simulink model "NIELITCombined_fixed"  (R2025a)
settings: Solver=ode45  StartTime=0.0  StopTime=100  MaxStep=2e-5  RelTol=1e-3
libraries: simulink x1
settings Model: Creator=naray  LastModifiedBy=naray

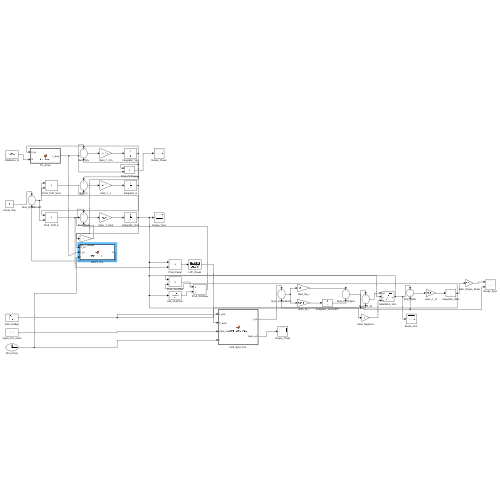
[thumbnail: Simulink's stored preview of the top-level diagram]
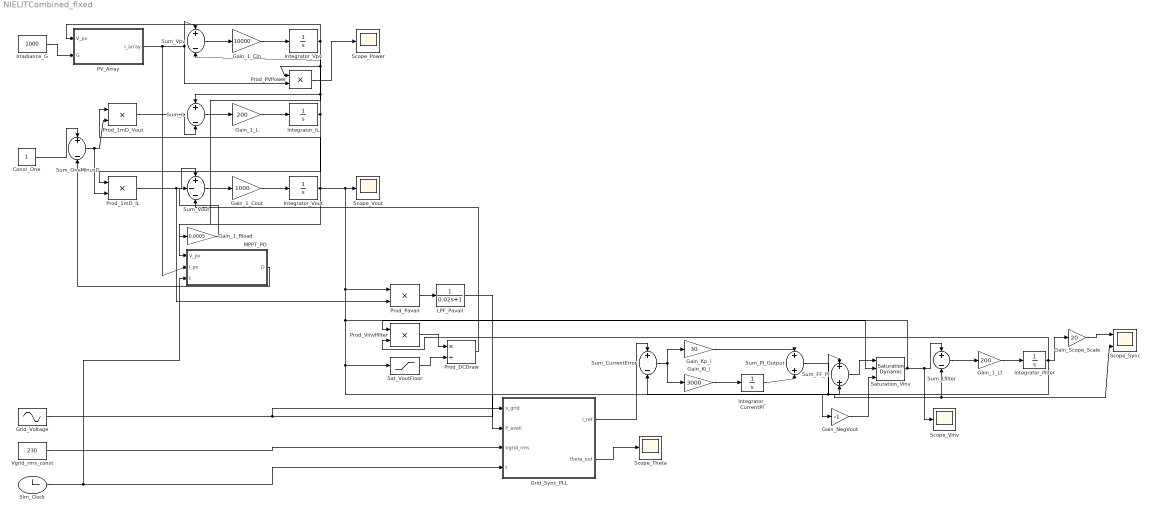
== system NIELITCombined_fixed ==
  Const_One : Constant
  Gain_1_Cin : Gain  Gain=10000
  Gain_1_Cout : Gain  Gain=1000
  Gain_1_L : Gain  Gain=200
  Gain_1_Lf : Gain  Gain=200
  Gain_1_Rload : Gain  Gain=0.0005
  Gain_Ki_i : Gain  Gain=3000
  Gain_Kp_i : Gain  Gain=30
  Gain_NegVout : Gain  Gain=-1
  Gain_Scope_Scale : Gain  Gain=20
  Grid_Sync_PLL : MATLAB Function  TreatAsAtomicUnit=on
  Grid_Voltage : Sin  Amplitude=325.2691  Frequency=314.1593  SampleTime=0
  Integrator_CurrentPI : Integrator
  Integrator_Vout : Integrator  InitialCondition=350
  Integrator_Vpv : Integrator  InitialCondition=300
  Integrator_iL : Integrator
  Integrator_ifilter : Integrator
  Irradiance_G : Constant  Value=1000
  LPF_Pavail : TransferFcn  Denominator=[0.02 1]
  MPPT_PO : MATLAB Function  TreatAsAtomicUnit=on
  PV_Array : MATLAB Function  TreatAsAtomicUnit=on
  Prod_1mD_Vout : Product
  Prod_1mD_iL : Product
  Prod_DCDraw : Product  Inputs=*/
  Prod_PVPower : Product
  Prod_Pavail : Product
  Prod_VinvIfilter : Product
  Sat_VoutFloor : Saturate  UpperLimit=1000  LowerLimit=50
  Saturation_Vinv : simulink/Discontinuities/Saturation Dynamic  OutMin=[]  OutMax=[]  OutDataTypeStr=Inherit: Same as second input  OutDataType=fixdt(1, 16)  OutScaling=2^-10  DoSatur=off
  Scope_Power : Scope
      settings: ActiveDisplayYMinimum=83.879513740278981  ActiveDisplayYMaximum=3287.1437398474195
  Scope_Sync : Scope  NumInputPorts=2
      settings: ActiveDisplayYMinimum=-448.184779047426  ActiveDisplayYMaximum=337.89270833968885
  Scope_Theta : Scope
      settings: ActiveDisplayYMinimum=-0.7853974821483809  ActiveDisplayYMaximum=7.0685802525916088
  Scope_Vinv : Scope
      settings: ActiveDisplayYMinimum=-415.88461066533625  ActiveDisplayYMaximum=415.4691551949615
  Scope_Vout : Scope
      settings: ActiveDisplayYMinimum=-1  ActiveDisplayYMaximum=1
  Sim_Clock : Clock
  Sum_CurrentError : Sum  Inputs=+-
  Sum_FF_PI : Sum
  Sum_Lfilter : Sum  Inputs=+-
  Sum_OneMinusD : Sum  Inputs=+-
  Sum_PI_Output : Sum
  Sum_Vout : Sum  Inputs=+--
  Sum_Vpv : Sum  Inputs=+-
  Sum_iL : Sum  Inputs=+-
  Vgrid_rms_const : Constant  Value=230
  wires:
  Irradiance_G/1 -> PV_Array/2(G)
  Integrator_Vpv/1 -> Sum_iL/1, MPPT_PO/1(V_pv), Prod_PVPower/1, PV_Array/1(V_pv)
  PV_Array/1(I_array) -> Sum_Vpv/1, Prod_PVPower/2, MPPT_PO/2(I_pv)
  Prod_PVPower/1 -> Scope_Power/1
  Integrator_iL/1 -> Sum_Vpv/2, Prod_1mD_iL/1
  Sum_Vpv/1 -> Gain_1_Cin/1
  Gain_1_Cin/1 -> Integrator_Vpv/1
  Prod_1mD_Vout/1 -> Sum_iL/2
  Sum_iL/1 -> Gain_1_L/1
  Gain_1_L/1 -> Integrator_iL/1
  Integrator_Vout/1 -> Gain_NegVout/1, Sat_VoutFloor/1, Saturation_Vinv/2, Prod_Pavail/1, Scope_Vout/1, Prod_1mD_Vout/1, Gain_1_Rload/1
  Sum_OneMinusD/1 -> Prod_1mD_Vout/2, Prod_1mD_iL/2
  Const_One/1 -> Sum_OneMinusD/1
  MPPT_PO/1(D) -> Sum_OneMinusD/2
  Prod_1mD_iL/1 -> Sum_Vout/1, Prod_Pavail/2
  Gain_1_Rload/1 -> Sum_Vout/2
  Prod_DCDraw/1 -> Sum_Vout/3
  Sum_Vout/1 -> Gain_1_Cout/1
  Gain_1_Cout/1 -> Integrator_Vout/1
  Grid_Voltage/1 -> Sum_Lfilter/2, Scope_Sync/2, Sum_FF_PI/1, Grid_Sync_PLL/1(v_grid)
  Prod_Pavail/1 -> LPF_Pavail/1
  LPF_Pavail/1 -> Grid_Sync_PLL/2(P_avail)
  Vgrid_rms_const/1 -> Grid_Sync_PLL/3(Vgrid_rms)
  Sim_Clock/1 -> Grid_Sync_PLL/4(t), MPPT_PO/3(t)
  Grid_Sync_PLL/1(i_ref) -> Sum_CurrentError/1
  Grid_Sync_PLL/2(theta_out) -> Scope_Theta/1
  Integrator_ifilter/1 -> Sum_CurrentError/2, Gain_Scope_Scale/1, Prod_VinvIfilter/2
  Sum_CurrentError/1 -> Gain_Kp_i/1, Gain_Ki_i/1
  Gain_Ki_i/1 -> Integrator_CurrentPI/1
  Gain_Kp_i/1 -> Sum_PI_Output/1
  Integrator_CurrentPI/1 -> Sum_PI_Output/2
  Sum_PI_Output/1 -> Sum_FF_PI/2
  Sum_FF_PI/1 -> Saturation_Vinv/1
  Gain_NegVout/1 -> Saturation_Vinv/3
  Saturation_Vinv/1 -> Scope_Vinv/1, Sum_Lfilter/1, Prod_VinvIfilter/1
  Sum_Lfilter/1 -> Gain_1_Lf/1
  Gain_1_Lf/1 -> Integrator_ifilter/1
  Gain_Scope_Scale/1 -> Scope_Sync/1
  Prod_VinvIfilter/1 -> Prod_DCDraw/1
  Sat_VoutFloor/1 -> Prod_DCDraw/2

== matlab function NIELITCombined_fixed/MPPT_PO ==
  settings: updateMethod=DISCRETE
  data: V_pv input; D output; I_pv input; t input
function D = MPPT_PO(V_pv, I_pv, t)
    persistent D_prev direction P_prev t_last
    if isempty(D_prev)
        D_prev = 0.5;      % your existing initial duty cycle
        direction = 1;
        P_prev = 0;
        t_last = -Inf;
    end

    Ts_mppt = 0.02;        % sample interval: ~4x the 20ms LPF time constant
    Dstep   = 0.005;       % consider halving your current step size too

    if (t - t_last) >= Ts_mppt
        P = V_pv * I_pv;
        if P < P_prev
            direction = -direction;
        end
        D_prev = D_prev + direction * Dstep;
        D_prev = min(max(D_prev, 0.05), 0.95);  % keep your existing D_min/D_max
        P_prev = P;
        t_last = t;
    end

    D = D_prev;   % hold last decision between updates
end

== matlab function NIELITCombined_fixed/PV_Array ==
  data: V_pv input; I_array output; G input
function I_array = PV_Array(V_pv, G)
% Simplified single-diode PV model for a 12-panel series STRING
Isc = 8.8; Voc = 444; n = 1.3; Ns = 720; Vt = 0.02585;
Iph = Isc * (G/1000);
Io  = Isc / (exp(Voc/(n*Vt*Ns)) - 1);
I_array = Iph - Io*(exp(V_pv/(n*Vt*Ns)) - 1);
I_array = max(I_array, 0);
end

== matlab function NIELITCombined_fixed/Grid_Sync_PLL ==
  settings: updateMethod=DISCRETE
  data: v_grid input; i_ref output; P_avail input; Vgrid_rms input; t input; theta_out output
function [i_ref, theta_out] = Grid_Sync_PLL(v_grid, P_avail, Vgrid_rms, t)
% SOGI-PLL (clock-based adaptive timing, vd-driven PI)
persistent x1 x2 theta integral_term t_prev
if isempty(x1)
    x1 = 0; x2 = 0; theta = 0; integral_term = 0; t_prev = 0;
end
dt = t - t_prev;
t_prev = t;
if dt <= 0
    dt = 1e-6;
end
k = 1.4142;
omega0 = 2*pi*50;
Kp_pll = 180;
Ki_pll = 3200;

x1_new = x1 + dt*omega0*(k*(v_grid - x1) - x2);
x2_new = x2 + dt*omega0*x1;
x1 = x1_new;
x2 = x2_new;

vd =  x1*cos(theta) + x2*sin(theta);
vq = -x1*sin(theta) + x2*cos(theta);

integral_term = integral_term + dt*Ki_pll*vd;
domega = Kp_pll*vd + integral_term;
omega = omega0 + domega;

theta = theta + dt*omega;
theta = mod(theta, 2*pi);
theta_out = theta;

I_ref_amplitude = (P_avail / Vgrid_rms) * sqrt(2);
i_ref = I_ref_amplitude * sin(theta);
end
